simulink model "lab1simulink"  (R2026b)
settings: Solver=FixedStepAuto  StopTime=0.02  FixedStep=0.0002
settings Model: Creator=ilqar  LastModifiedBy=ilqar

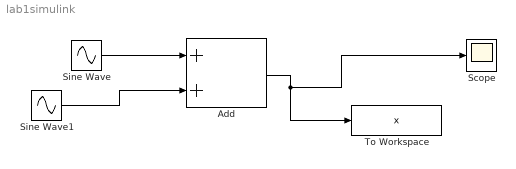
== system lab1simulink ==
  Add : Sum
  Scope : Scope
      settings: ActiveDisplayYMinimum=-2.4612215945469318  ActiveDisplayYMaximum=2.2829055631174882
  Sine Wave : Sin  Frequency=2*pi*100  Phase=0.5*pi  SampleTime=0
  Sine Wave1 : Sin  Frequency=2*pi*200  Phase=0.5*pi  SampleTime=0
  To Workspace : ToWorkspace  VariableName=x  SampleTime=-1
  wires:
  Sine Wave/1 -> Add/1
  Sine Wave1/1 -> Add/2
  Add/1 -> To Workspace/1, Scope/1
